simulink model "lab6_task2"  (R2024b)
settings: Solver=ode45  StartTime=0.0  StopTime=5.0  MaxStep=0.01  RelTol=1e-3
settings Model: Creator=Beanie  LastModifiedBy=Beanie

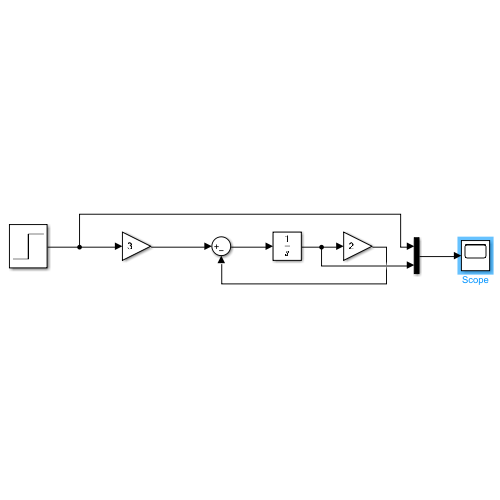
[thumbnail: Simulink's stored preview of the top-level diagram]
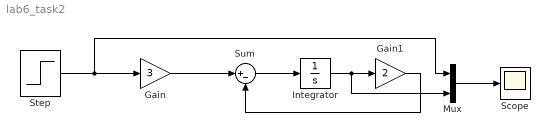
== system lab6_task2 ==
  Gain : Gain  Gain=3
  Gain1 : Gain  Gain=2
  Integrator : Integrator  InitialCondition=1
  Mux : Mux  Inputs=2
  Scope : Scope
  Step : Step  Time=0  After=2  SampleTime=0
  Sum : Sum  Inputs=|+-
  wires:
  Sum/1 -> Integrator/1
  Mux/1 -> Scope/1
  Gain/1 -> Sum/1
  Step/1 -> Mux/1, Gain/1
  Gain1/1 -> Sum/2
  Integrator/1 -> Mux/2, Gain1/1
